simulink model "PMSM"  (R2024a)
settings: Solver=VariableStepAuto  StartTime=0.0  StopTime=1  RelTol=1e-3
InitFcn:
  | Ts = 1e-6;
  | Ts_pwm = 1/20e3;
  | dead_time=0;
  | R = 0.559;
  | Ld = 4.24e-3;
  | Lq = 4.24e-3;
  | Laa=2.83e-3
  | Pn = 4;
  | flux = 0.339;
  | Vdc=400
undefined symbols (not defined in the file): DiscIntNeverNeededParam
libraries: spsIGBTDiodeLib x6, powerlib_extras x2, spsPermanentMagnetSynchronousMachineLib x1, simulink x1, spsDCVoltageSourceLib x1, spsCurrentMeasurementLib x1, spsVoltageMeasurementLib x1, sps_lib x1
settings Model: Creator=16199  LastModifiedBy=16685
settings SolverCC: AlgebraicLoopSolver=TrustRegion
settings DataIOCC: ReturnWorkspaceOutputs=off
settings DebuggingCC: UnconnectedInputMsg=warning  UnconnectedOutputMsg=warning  UnconnectedLineMsg=warning  ArithmeticOperatorsInVariantConditions=warning
settings ModelReferenceCC: EnableRefExpFcnMdlSchedulingChecks=on
settings SFSimCC: CustomCodeUndefinedFunction=UseInterfaceOnly
settings RTWCC: GPUComputeCapability=3.5

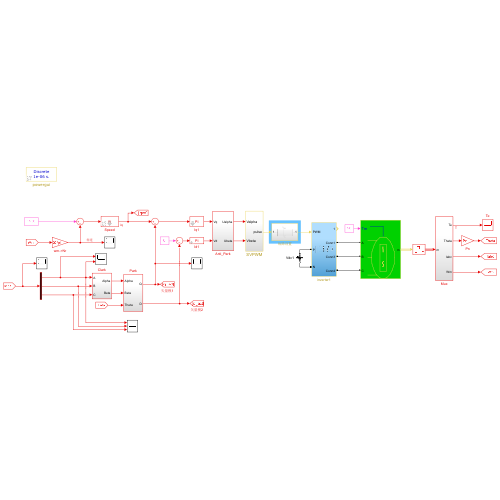
[thumbnail: Simulink's stored preview of the top-level diagram]
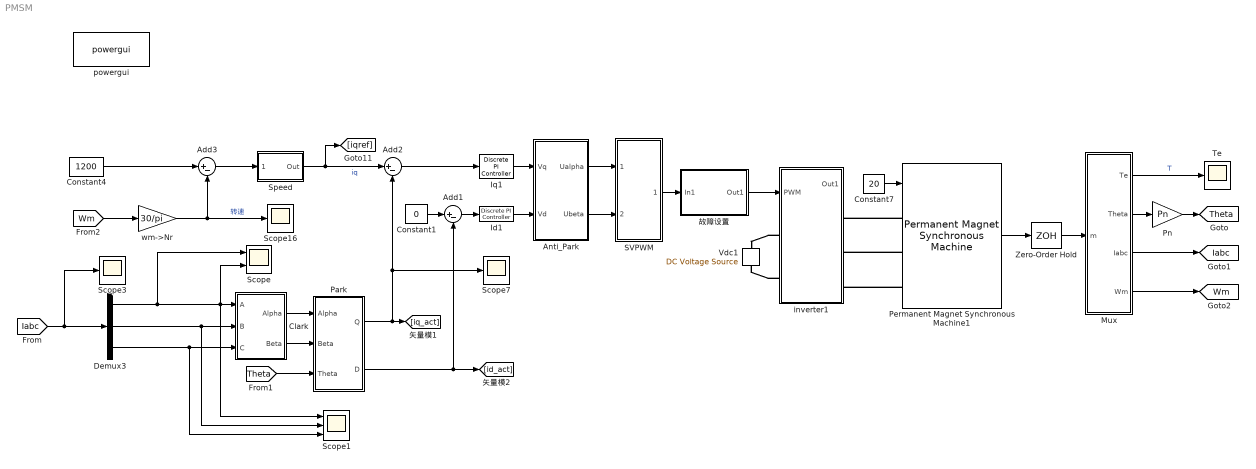
== system PMSM ==
  Add1 : Sum  Inputs=|+-
  Add2 : Sum  Inputs=|+-
  Add3 : Sum  Inputs=|+-
  Anti_Park : Subsystem
  Clark : Subsystem
  Constant1 : Constant  Value=0
  Constant4 : Constant  Value=1200
  Constant7 : Constant  Value=20
  Demux3 : Demux  Outputs=3
  Id1 : powerlib_extras/Discrete  Control Blocks/Discrete PI Controller  Kp=Ld*552*4  Ki=R*552*1  Par_Limits=[Vdc*0.9*sqrt(1/3) -Vdc*0.9*sqrt(1/3)]  Init=0  Ts=Ts
  Iq1 : powerlib_extras/Discrete  Control Blocks/Discrete PI Controller  Kp=Lq*552*4  Ki=R*552*1  Par_Limits=[Vdc*0.9*sqrt(1/3) -Vdc*0.9*sqrt(1/3)]  Init=0  Ts=Ts
  Mux : Subsystem
  Park : Subsystem
  Permanent Magnet Synchronous Machine1 : spsPermanentMagnetSynchronousMachineLib/Permanent Magnet Synchronous Machine  NbPhases=3  FluxDistribution=Sinusoidal  RotorType=Round  MechanicalLoad=Torque Tm  PresetModel=No  ShowDetailedParameters=on  MeasurementBus=off  Resistance=0.559  Inductance=8.5e-3  dqInductances=[5.25e-3,12e-3]  La=4.24e-3  MachineConstant=Flux linkage established by magnets (V.s)  Flux=0.339  VoltageCst=245.9512  TorqueCst=2.034  Flat=120  Mechanical=[0.00406 0.008 4 0]  PolePairs=3  InitialConditions=[0,0, 0,0]  InitialConditions5ph=[0 0 0 0 0 0]  RefAngle=Aligned with phase A axis (original Park)  IterativeDiscreteModel=Trapezoidal non iterative  TsBlock=-1  TsPowergui=0
  Pn : Gain  Gain=Pn
  SVPWM : Subsystem
  Scope : Scope  NumInputPorts=2
  Scope1 : Scope  NumInputPorts=3
  Scope16 : Scope
  Scope3 : Scope
  Scope7 : Scope
  Speed : Subsystem  AncestorBlock=|  DialogController=POWERSYS.PowerSysDialog  mask(Discrete PI Controller){Kpw=0.108, Kiw=4, Ba=0.1, Par_Limits=[100 -100], Init=0, Ts=Ts}
      | powerlib_extras/Discrete 
      | Control Blocks/Discrete
      | PI Controller
      mask prompts: Kpw "Proportional gain (Kp):"; Kiw "Integral gain (Ki):"; Ba "feedback gain (Ba)"; Par_Limits "Output limits: [ Upper   Lower ]"; Init "Output initial value:"; Ts "Sample time:"
      mask help: This block implements a discrete PI controller.
      mask init:
      | UpperLimit=Par_Limits(1);
      | LowerLimit=Par_Limits(2);
      | power_initmask();
      mask Help: This block is part of a subset of blocks in the Extras library that does not have documentation associated with it, other than the block mask description.
      mask Display: disp('PI');
  Te : Scope
  Vdc1 : spsDCVoltageSourceLib/DC Voltage Source  Amplitude=Vdc  Measurements=None
  Zero-Order Hold : ZeroOrderHold  SampleTime=2e-6
  inverter1 : Subsystem
  powergui : sps_lib/powergui  SimulationMode=Discrete  SampleTime=Ts  frequency=60  Iterations=50  frequencyindice=0  Pbase=100e6  ErrMax=1e-4  UnitsV=kV  UnitsW=MW  buscounter=0  FunctionMessages=off  echomessages=off  EnableUseOfTLC=off  CurrentSourceSwitches=off  DisableSnubberDevices=off  DisableRonSwitches=off  DisableVfSwitches=off  DisplayEquations=off  AutomaticDiscreteSolvers=off  SolverType=Tustin/Backward Euler (TBE)  Interpol=off  ExternalGateDelay=off  methode=off  Ts=100  x0status=blocks  SPID=off  SwTol=0  HookPort=off  NonlinearTolerance=1e-4  nMaxIteration=100  ContinueOnMaxIteration=off  RestoreLinks=warning  ResistiveCurrentMeasurement=off  Frange=[0:2:500]  Ylog=off  Xlog=on  ShowGrid=off  save=off  variable=ZData  structure=ScopeData3  ZoomFFT=off  StartTime=0.4  cycles=1  DisplayStyle=1  fundamental=62  FreqAxis=off  MaxFrequency=1000  frequencyindicesteady=1  RmsSteady=1  display=off
  wm->Nr : Gain  Gain=30/pi
  故障设置 : Subsystem
  tag scope: Iabc=global, Theta=global, Wm=global
  wires:
  Demux3/1 -> Scope/2, Scope1/1, Clark/1(A), Scope/1
  Clark/2(Beta) -> Park/2(Beta)
  Demux3/3 -> Scope1/3, Clark/3(C)
  Constant7/1 -> Permanent Magnet Synchronous Machine1/1
  Mux/1(Te) -> Te/1  "T"
  Add2/1 -> Iq1/1
  [Wm] -> wm->Nr/1
  Anti_Park/1(Ualpha) -> SVPWM/1(Valpha)
  Demux3/2 -> Scope1/2, Clark/2(B)
  Pn/1 -> [Theta]
  SVPWM/1(pulse) -> 故障设置/1(In1)
  Clark/1(Alpha) -> Park/1(Alpha)
  Iq1/1 -> Anti_Park/1(Vq)
  Park/1(Q) -> Scope7/1, Add2/2, [iq_act]
  Add1/1 -> Id1/1
  [Iabc] -> Demux3/1, Scope3/1
  Add3/1 -> Speed/1(Error)
  [Theta] -> Park/3(Theta)
  Anti_Park/2(Ubeta) -> SVPWM/2(Vbeta)
  Speed/1(Out) -> Add2/1, [iqref]  "iq"
  故障设置/1(Out1) -> inverter1/1(PWM)
  Constant4/1 -> Add3/1
  Park/2(D) -> Add1/2, [id_act]
  Zero-Order Hold/1 -> Mux/1(m)
  wm->Nr/1 -> Add3/2, Scope16/1  "转速"
  Constant1/1 -> Add1/1
  Mux/3(Iabc) -> [Iabc]
  Id1/1 -> Anti_Park/2(Vd)
  Mux/4(Wm) -> [Wm]
  Mux/2(Theta) -> Pn/1
  Permanent Magnet Synchronous Machine1/1 -> Zero-Order Hold/1
  connections:
  Permanent Magnet Synchronous Machine1/LConn2 -- inverter1/RConn2
  inverter1/LConn1 -- Vdc1/RConn1
  Permanent Magnet Synchronous Machine1/LConn1 -- inverter1/RConn1
  inverter1/LConn2 -- Vdc1/LConn1
  Permanent Magnet Synchronous Machine1/LConn3 -- inverter1/RConn3

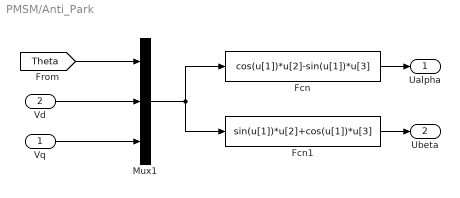
== system PMSM/Anti_Park ==
  Vq : Inport
  Vd : Inport  Port=2
  Fcn : Fcn  Expr=cos(u[1])*u[2]-sin(u[1])*u[3]
  Fcn1 : Fcn  Expr=sin(u[1])*u[2]+cos(u[1])*u[3]
  Mux1 : Mux  Inputs=3
  Ualpha : Outport
  Ubeta : Outport  Port=2
  wires:
  Fcn1/1 -> Ubeta/1
  Fcn/1 -> Ualpha/1
  Mux1/1 -> Fcn/1, Fcn1/1
  Vd/1 -> Mux1/2
  Vq/1 -> Mux1/3
  [Theta] -> Mux1/1

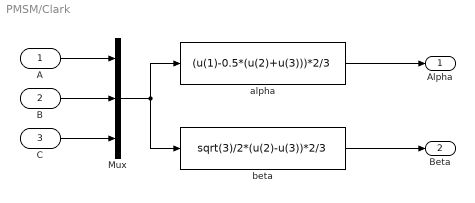
== system PMSM/Clark ==
  A : Inport
  B : Inport  Port=2
  C : Inport  Port=3
  Mux : Mux  Inputs=3
  alpha : Fcn  Expr=(u(1)-0.5*(u(2)+u(3)))*2/3
  beta : Fcn  Expr=sqrt(3)/2*(u(2)-u(3))*2/3
  Alpha : Outport
  Beta : Outport  Port=2
  wires:
  alpha/1 -> Alpha/1
  B/1 -> Mux/2
  C/1 -> Mux/3
  A/1 -> Mux/1
  Mux/1 -> beta/1, alpha/1
  beta/1 -> Beta/1

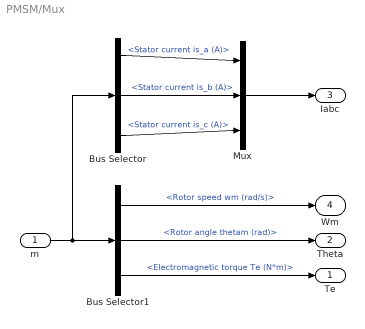
== system PMSM/Mux ==
  m : Inport
  Bus Selector : BusSelector  OutputSignals=Stator current is_a (A),Stator current is_b (A),Stator current is_c (A)
  Bus Selector1 : BusSelector  OutputSignals=Rotor speed wm (rad/s),Rotor angle thetam (rad),Electromagnetic torque Te (N*m)
  Mux : Mux  Inputs=3
  Te : Outport
  Theta : Outport  Port=2
  Iabc : Outport  Port=3
  Wm : Outport  Port=4
  wires:
  Bus Selector1/1 -> Wm/1  "<Rotor speed wm (rad/s)>"
  Bus Selector1/2 -> Theta/1  "<Rotor angle thetam (rad)>"
  Bus Selector1/3 -> Te/1  "<Electromagnetic torque Te (N*m)>"
  m/1 -> Bus Selector/1, Bus Selector1/1
  Bus Selector/2 -> Mux/2  "<Stator current is_b (A)>"
  Bus Selector/3 -> Mux/3  "<Stator current is_c (A)>"
  Bus Selector/1 -> Mux/1  "<Stator current is_a (A)>"
  Mux/1 -> Iabc/1

== system PMSM/Park ==
  Alpha : Inport
  Beta : Inport  Port=2
  Theta : Inport  Port=3
  Mux : Mux  Inputs=3
  d : Fcn  Expr=u(1)*cos(u(3))+u(2)*sin(u(3))
  q : Fcn  Expr=-u(1)*sin(u(3))+u(2)*cos(u(3))
  Q : Outport
  D : Outport  Port=2
  wires:
  d/1 -> D/1
  Beta/1 -> Mux/2
  Alpha/1 -> Mux/1
  Mux/1 -> d/1, q/1
  q/1 -> Q/1
  Theta/1 -> Mux/3

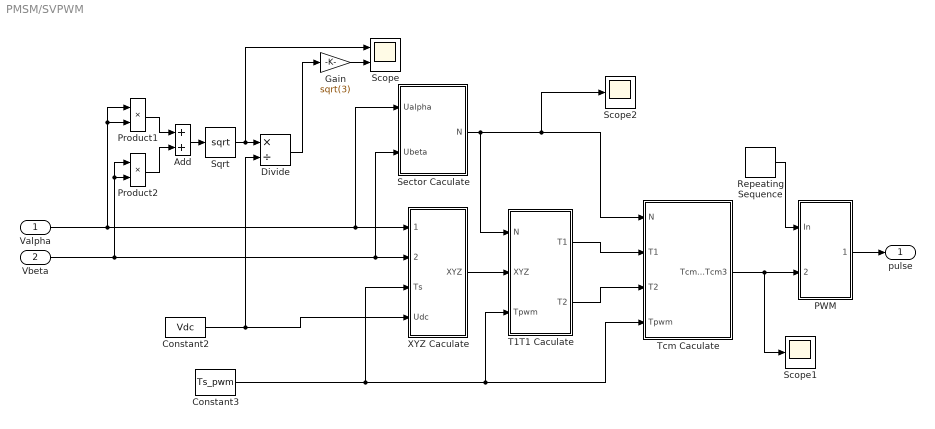
== system PMSM/SVPWM ==
  Valpha : Inport
  Vbeta : Inport  Port=2
  Add : Sum
  Constant2 : Constant  Value=Vdc
  Constant3 : Constant  Value=Ts_pwm
  Divide : Product  Inputs=*/
  Gain : Gain  Gain=sqrt(3)
  PWM : Subsystem
  Product1 : Product  RndMeth=Zero
  Product2 : Product  RndMeth=Zero
  Repeating Sequence : simulink/Sources/Repeating Sequence  rep_seq_t=[0 0.5*Ts_pwm Ts_pwm]  rep_seq_y=[0 0.5*Ts_pwm 0]
  Scope : Scope  NumInputPorts=2
  Scope1 : Scope
  Scope2 : Scope
  Sector Caculate : Subsystem
  Sqrt : Sqrt
  T1T1 Caculate : Subsystem
  Tcm Caculate : Subsystem
  XYZ Caculate : Subsystem
  pulse : Outport  VectorParamsAs1DForOutWhenUnconnected=off
  wires:
  PWM/1(PWM) -> pulse/1
  Repeating Sequence/1 -> PWM/1(In)
  Vbeta/1 -> Product2/2, Product2/1, XYZ Caculate/2(Ubeta), Sector Caculate/2(Ubeta)
  T1T1 Caculate/1(T1) -> Tcm Caculate/2(T1)
  Valpha/1 -> Product1/2, Product1/1, XYZ Caculate/1(Ualpha), Sector Caculate/1(Ualpha)
  T1T1 Caculate/2(T2) -> Tcm Caculate/3(T2)
  Sector Caculate/1("N ") -> Scope2/1, Tcm Caculate/1(N), T1T1 Caculate/1(N)
  XYZ Caculate/1(XYZ) -> T1T1 Caculate/2(XYZ)
  Constant3/1 -> XYZ Caculate/3(Ts), Tcm Caculate/4(Tpwm), T1T1 Caculate/3(Tpwm)
  Constant2/1 -> XYZ Caculate/4(Udc), Divide/2
  Tcm Caculate/1(Tcm1 Tcm2 Tcm3) -> Scope1/1, PWM/2(Tcm123)
  Product1/1 -> Add/1
  Product2/1 -> Add/2
  Add/1 -> Sqrt/1
  Sqrt/1 -> Scope/1, Divide/1
  Divide/1 -> Gain/1
  Gain/1 -> Scope/2

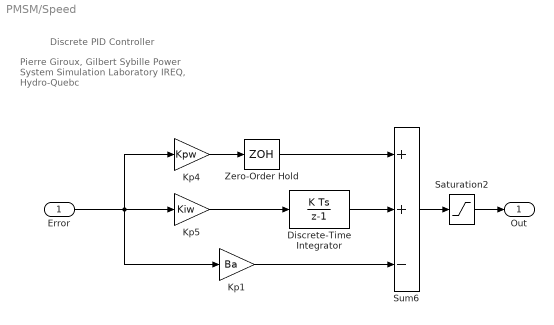
== system PMSM/Speed ==
  note: Discrete PID Controller
  note: Pierre Giroux, Gilbert Sybille
      | Power System Simulation Laboratory
      | IREQ, Hydro-Quebc
  Error : Inport  SampleTime=Ts
  Discrete-Time Integrator : DiscreteIntegrator  InitialCondition=Init  SampleTime=Ts  LimitOutput=on  UpperSaturationLimit=UpperLimit  LowerSaturationLimit=LowerLimit  ICPrevOutput=DiscIntNeverNeededParam  ICPrevScaledInput=DiscIntNeverNeededParam
  Kp1 : Gain  Gain=Ba  SaturateOnIntegerOverflow=on  SampleTime=Ts  OutDataTypeStr=Inherit: Same as input  ParamDataTypeStr=Inherit: Same as input
  Kp4 : Gain  Gain=Kpw  SaturateOnIntegerOverflow=on  SampleTime=Ts  OutDataTypeStr=Inherit: Same as input  ParamDataTypeStr=Inherit: Same as input
  Kp5 : Gain  Gain=Kiw  SaturateOnIntegerOverflow=on  SampleTime=Ts  OutDataTypeStr=Inherit: Same as input  ParamDataTypeStr=Inherit: Same as input
  Saturation2 : Saturate  UpperLimit=UpperLimit  LowerLimit=LowerLimit  SampleTime=Ts
  Sum6 : Sum  Inputs=++-  InputSameDT=on  SaturateOnIntegerOverflow=on  SampleTime=Ts  OutDataTypeStr=Inherit: Same as first input
  Zero-Order Hold : ZeroOrderHold  SampleTime=Ts
  Out : Outport  SampleTime=Ts  InitialOutput=0
  wires:
  Error/1 -> Kp1/1, Kp5/1, Kp4/1
  Zero-Order Hold/1 -> Sum6/1
  Saturation2/1 -> Out/1
  Discrete-Time Integrator/1 -> Sum6/2
  Kp4/1 -> Zero-Order Hold/1
  Kp5/1 -> Discrete-Time Integrator/1
  Sum6/1 -> Saturation2/1
  Kp1/1 -> Sum6/3

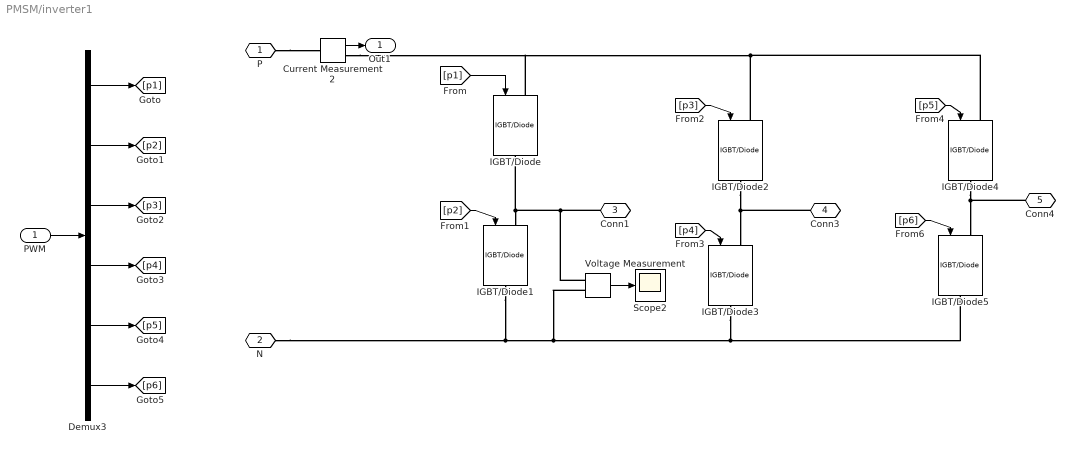
== system PMSM/inverter1 ==
  PWM : Inport
  Current Measurement2 : spsCurrentMeasurementLib/Current Measurement  PhasorSimulation=off  OutputType=Complex  PSBequivalent=0
  Demux3 : Demux  Outputs=6
  IGBT/Diode{,1..5} (6 alike) : spsIGBTDiodeLib/IGBT//Diode  Ron=1e-3  Rs=1e5  Cs=inf  Measurements=off
  Scope2 : Scope
  Voltage Measurement : spsVoltageMeasurementLib/Voltage Measurement  PhasorSimulation=off  OutputType=Complex  PSBequivalent=0
  P : PMIOPort  Side=Left
  N : PMIOPort  Port=2  Side=Left
  Conn1 : PMIOPort  Port=3  Side=Right
  Conn3 : PMIOPort  Port=4  Side=Right
  Conn4 : PMIOPort  Port=5  Side=Right
  Out1 : Outport  VectorParamsAs1DForOutWhenUnconnected=off
  wires:
  [p6] -> IGBT/Diode5/1
  [p3] -> IGBT/Diode2/1
  [p4] -> IGBT/Diode3/1
  [p2] -> IGBT/Diode1/1
  [p5] -> IGBT/Diode4/1
  PWM/1 -> Demux3/1
  Demux3/2 -> [p2]
  Demux3/3 -> [p3]
  Demux3/4 -> [p4]
  Demux3/5 -> [p5]
  Demux3/6 -> [p6]
  [p1] -> IGBT/Diode/1
  Current Measurement2/1 -> Out1/1
  Voltage Measurement/1 -> Scope2/1
  Demux3/1 -> [p1]
  connections:
  Conn1/RConn1 -- IGBT/Diode/RConn1 -- IGBT/Diode1/LConn1 -- Voltage Measurement/LConn1
  IGBT/Diode4/RConn1 -- Conn4/RConn1 -- IGBT/Diode5/LConn1
  IGBT/Diode2/RConn1 -- Conn3/RConn1 -- IGBT/Diode3/LConn1
  IGBT/Diode2/LConn1 -- IGBT/Diode/LConn1 -- Current Measurement2/RConn1 -- IGBT/Diode4/LConn1
  N/RConn1 -- Voltage Measurement/LConn2 -- IGBT/Diode3/RConn1 -- IGBT/Diode5/RConn1 -- IGBT/Diode1/RConn1
  P/RConn1 -- Current Measurement2/LConn1

== system PMSM/故障设置 ==
  In1 : Inport
  Demux1 : Demux  Outputs=6
  Mux1 : Mux  Inputs=6
  Product : Product
  Product1 : Product
  Step : Step  Time=0.5  Before=1  After=0  SampleTime=0
  Out1 : Outport  VectorParamsAs1DForOutWhenUnconnected=off
  wires:
  Mux1/1 -> Out1/1
  In1/1 -> Demux1/1
  Step/1 -> Product1/1, Product/1
  Demux1/5 -> Mux1/5
  Demux1/4 -> Mux1/4
  Demux1/3 -> Mux1/3
  Demux1/6 -> Mux1/6
  Demux1/1 -> Mux1/1
  Demux1/2 -> Mux1/2

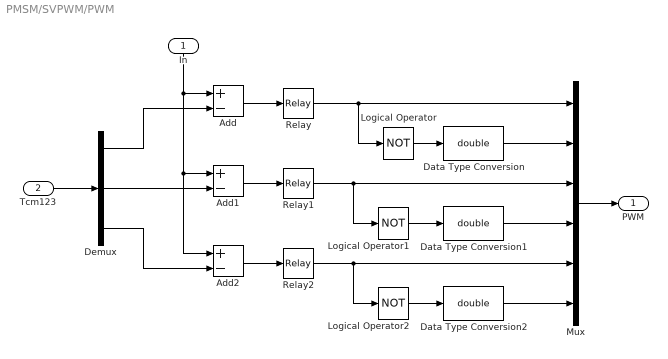
== system PMSM/SVPWM/PWM ==
  In : Inport
  Tcm123 : Inport  Port=2
  Add : Sum  Inputs=+-
  Add1 : Sum  Inputs=+-
  Add2 : Sum  Inputs=+-
  Data Type Conversion : DataTypeConversion  OutDataTypeStr=double  SaturateOnIntegerOverflow=off  RndMeth=Floor
  Data Type Conversion1 : DataTypeConversion  OutDataTypeStr=double  SaturateOnIntegerOverflow=off  RndMeth=Floor
  Data Type Conversion2 : DataTypeConversion  OutDataTypeStr=double  SaturateOnIntegerOverflow=off  RndMeth=Floor
  Demux : Demux  Outputs=3
  Logical Operator : Logic  Operator=NOT  AllPortsSameDT=off  OutDataTypeStr=boolean
  Logical Operator1 : Logic  Operator=NOT  AllPortsSameDT=off  OutDataTypeStr=boolean
  Logical Operator2 : Logic  Operator=NOT  AllPortsSameDT=off  OutDataTypeStr=boolean
  Mux : Mux  Inputs=6
  Relay : Relay  OffSwitchValue=-eps
  Relay1 : Relay  OffSwitchValue=-eps
  Relay2 : Relay  OffSwitchValue=-eps
  PWM : Outport  VectorParamsAs1DForOutWhenUnconnected=off
  wires:
  Demux/3 -> Add2/2
  Demux/2 -> Add1/2
  Demux/1 -> Add/2
  Relay2/1 -> Mux/5, Logical Operator2/1
  Relay1/1 -> Mux/3, Logical Operator1/1
  Relay/1 -> Logical Operator/1, Mux/1
  Mux/1 -> PWM/1
  Data Type Conversion/1 -> Mux/2
  Data Type Conversion1/1 -> Mux/4
  Data Type Conversion2/1 -> Mux/6
  Logical Operator2/1 -> Data Type Conversion2/1
  Logical Operator1/1 -> Data Type Conversion1/1
  Logical Operator/1 -> Data Type Conversion/1
  Add1/1 -> Relay1/1
  Add2/1 -> Relay2/1
  Add/1 -> Relay/1
  In/1 -> Add/1, Add2/1, Add1/1
  Tcm123/1 -> Demux/1

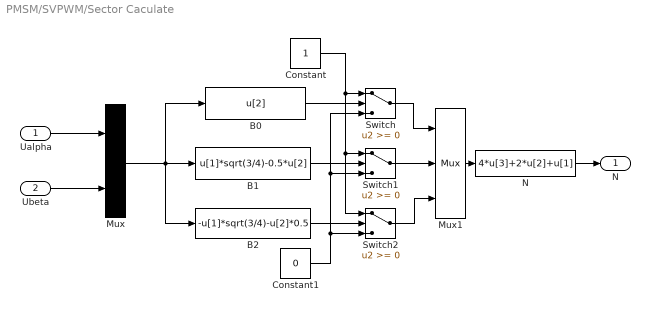
== system PMSM/SVPWM/Sector Caculate ==
  Ualpha : Inport
  Ubeta : Inport  Port=2
  B0 : Fcn  Expr=u[2]
  B1 : Fcn  Expr=u[1]*sqrt(3/4)-0.5*u[2]
  B2 : Fcn  Expr=-u[1]*sqrt(3/4)-u[2]*0.5
  Constant : Constant
  Constant1 : Constant  Value=0
  Mux : Mux  Inputs=2
  Mux1 : Mux  Inputs=3
  N : Fcn  Expr=4*u[3]+2*u[2]+u[1]
  Switch : Switch  SaturateOnIntegerOverflow=off  InputSameDT=off
  Switch1 : Switch  SaturateOnIntegerOverflow=off  InputSameDT=off
  Switch2 : Switch  SaturateOnIntegerOverflow=off  InputSameDT=off
  "N " : Outport  VectorParamsAs1DForOutWhenUnconnected=off
  wires:
  Switch2/1 -> Mux1/3
  Switch/1 -> Mux1/1
  Ualpha/1 -> Mux/1
  Ubeta/1 -> Mux/2
  Mux/1 -> B2/1, B1/1, B0/1
  B0/1 -> Switch/2
  B1/1 -> Switch1/2
  B2/1 -> Switch2/2
  Constant/1 -> Switch/1, Switch2/1, Switch1/1
  Constant1/1 -> Switch/3, Switch1/3, Switch2/3
  Switch1/1 -> Mux1/2
  Mux1/1 -> N/1
  N/1 -> "N "/1

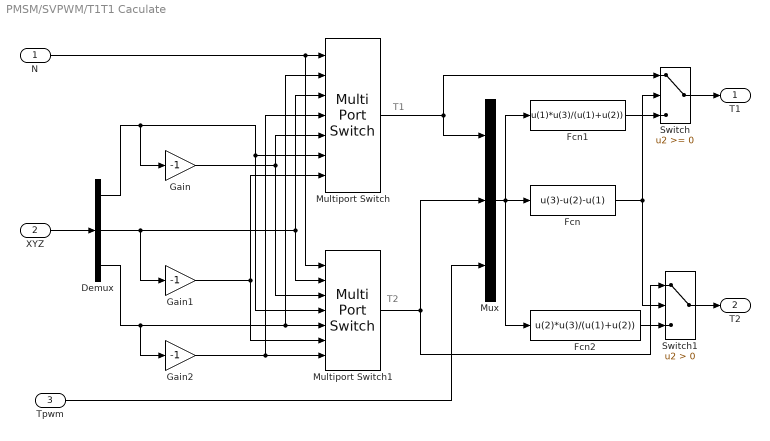
== system PMSM/SVPWM/T1T1 Caculate ==
  note: T1
  note: T2
  N : Inport
  XYZ : Inport  Port=2
  Tpwm : Inport  Port=3
  Demux : Demux  Outputs=3
  Fcn : Fcn  Expr=u(3)-u(2)-u(1)
  Fcn1 : Fcn  Expr=u(1)*u(3)/(u(1)+u(2))
  Fcn2 : Fcn  Expr=u(2)*u(3)/(u(1)+u(2))
  Gain : Gain  Gain=-1
  Gain1 : Gain  Gain=-1
  Gain2 : Gain  Gain=-1
  Multiport Switch : MultiPortSwitch  Inputs=6  SaturateOnIntegerOverflow=off  InputSameDT=off
  Multiport Switch1 : MultiPortSwitch  Inputs=6  SaturateOnIntegerOverflow=off  InputSameDT=off
  Mux : Mux  Inputs=3
  Switch : Switch  SaturateOnIntegerOverflow=off  InputSameDT=off
  Switch1 : Switch  Criteria=u2 > Threshold  SaturateOnIntegerOverflow=off  InputSameDT=off
  T1 : Outport  VectorParamsAs1DForOutWhenUnconnected=off
  T2 : Outport  Port=2  VectorParamsAs1DForOutWhenUnconnected=off
  wires:
  Tpwm/1 -> Mux/3
  XYZ/1 -> Demux/1
  Switch1/1 -> T2/1
  Switch/1 -> T1/1
  Fcn2/1 -> Switch1/3
  Fcn1/1 -> Switch/3
  Fcn/1 -> Switch/2, Switch1/2
  Mux/1 -> Fcn1/1, Fcn/1, Fcn2/1
  Multiport Switch/1 -> Switch/1, Mux/1
  Multiport Switch1/1 -> Switch1/1, Mux/2
  N/1 -> Multiport Switch/1, Multiport Switch1/1
  Demux/2 -> Multiport Switch/3, Multiport Switch1/2, Gain1/1
  Demux/3 -> Multiport Switch1/5, Multiport Switch/2, Gain2/1
  Demux/1 -> Multiport Switch/6, Multiport Switch1/4, Gain/1
  Gain/1 -> Multiport Switch1/3, Multiport Switch/5
  Gain2/1 -> Multiport Switch/4, Multiport Switch1/7
  Gain1/1 -> Multiport Switch1/6, Multiport Switch/7

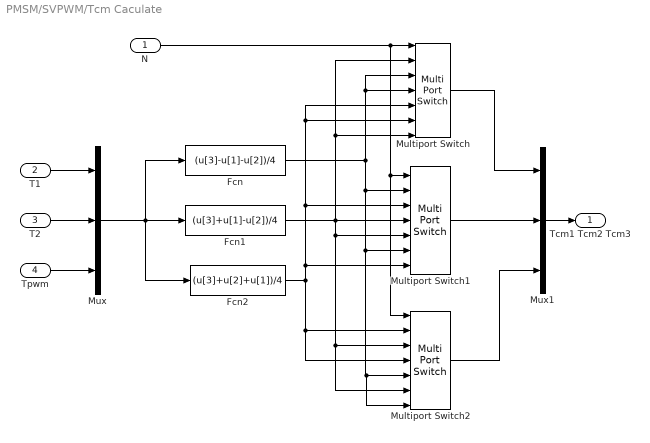
== system PMSM/SVPWM/Tcm Caculate ==
  N : Inport
  T1 : Inport  Port=2
  T2 : Inport  Port=3
  Tpwm : Inport  Port=4
  Fcn : Fcn  Expr=(u[3]-u[1]-u[2])/4
  Fcn1 : Fcn  Expr=(u[3]+u[1]-u[2])/4
  Fcn2 : Fcn  Expr=(u[3]+u[2]+u[1])/4
  Multiport Switch : MultiPortSwitch  Inputs=6  SaturateOnIntegerOverflow=off  InputSameDT=off
  Multiport Switch1 : MultiPortSwitch  Inputs=6  SaturateOnIntegerOverflow=off  InputSameDT=off
  Multiport Switch2 : MultiPortSwitch  Inputs=6  SaturateOnIntegerOverflow=off  InputSameDT=off
  Mux : Mux  Inputs=3
  Mux1 : Mux  Inputs=3
  Tcm1 Tcm2 Tcm3 : Outport  VectorParamsAs1DForOutWhenUnconnected=off
  wires:
  Mux/1 -> Fcn2/1, Fcn/1, Fcn1/1
  Tpwm/1 -> Mux/3
  T2/1 -> Mux/2
  T1/1 -> Mux/1
  Multiport Switch2/1 -> Mux1/3
  Multiport Switch1/1 -> Mux1/2
  Multiport Switch/1 -> Mux1/1
  Mux1/1 -> Tcm1 Tcm2 Tcm3/1
  Fcn/1 -> Multiport Switch/3, Multiport Switch/4, Multiport Switch1/6, Multiport Switch2/5, Multiport Switch2/7, Multiport Switch1/2
  Fcn1/1 -> Multiport Switch1/5, Multiport Switch2/3, Multiport Switch2/6, Multiport Switch1/4, Multiport Switch/7, Multiport Switch/2
  Fcn2/1 -> Multiport Switch/5, Multiport Switch/6, Multiport Switch1/3, Multiport Switch1/7, Multiport Switch2/2, Multiport Switch2/4
  N/1 -> Multiport Switch2/1, Multiport Switch1/1, Multiport Switch/1

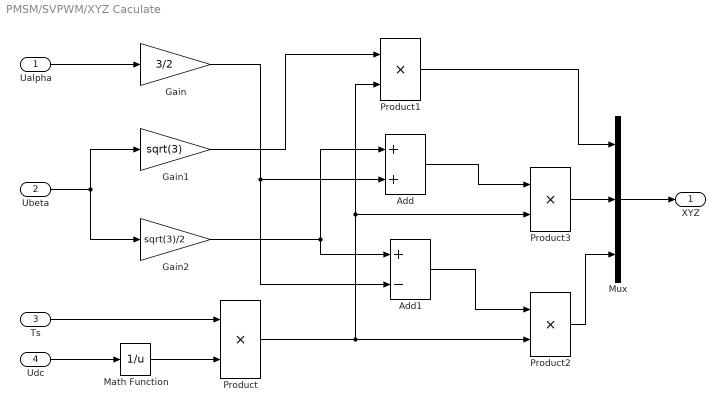
== system PMSM/SVPWM/XYZ Caculate ==
  Ualpha : Inport
  Ubeta : Inport  Port=2
  Ts : Inport  Port=3
  Udc : Inport  Port=4
  Add : Sum
  Add1 : Sum  Inputs=+-
  Gain : Gain  Gain=3/2
  Gain1 : Gain  Gain=sqrt(3)
  Gain2 : Gain  Gain=sqrt(3)/2
  Math Function : Math  Operator=reciprocal  SignedPower=on
  Mux : Mux  Inputs=3
  Product{,1..3} (4 alike) : Product  RndMeth=Zero
  XYZ : Outport  VectorParamsAs1DForOutWhenUnconnected=off
  wires:
  Mux/1 -> XYZ/1
  Product1/1 -> Mux/1
  Product3/1 -> Mux/2
  Product2/1 -> Mux/3
  Ualpha/1 -> Gain/1
  Ubeta/1 -> Gain2/1, Gain1/1
  Udc/1 -> Math Function/1
  Math Function/1 -> Product/2
  Ts/1 -> Product/1
  Gain1/1 -> Product1/1
  Product/1 -> Product2/2, Product1/2, Product3/2
  Gain/1 -> Add1/2, Add/2
  Gain2/1 -> Add/1, Add1/1
  Add1/1 -> Product2/1
  Add/1 -> Product3/1
